simulink model "rs_tlcd_predictive_control"  (R2026a)
settings: Solver=FixedStepDiscrete  StartTime=0  StopTime=pc_tstop  FixedStep=0.01
settings Model: Creator=cys  LastModifiedBy=cys
settings DebuggingCC: AlgebraicLoopMsg=error

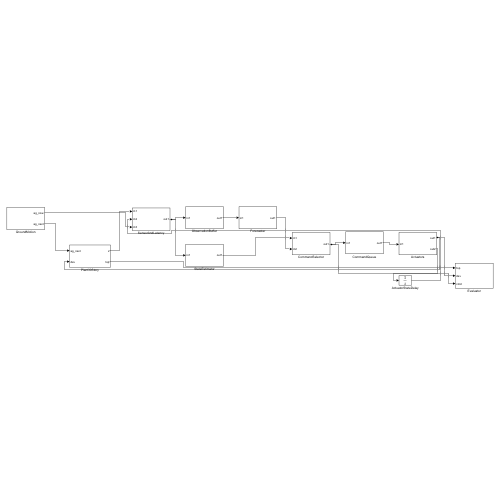
[thumbnail: Simulink's stored preview of the top-level diagram]
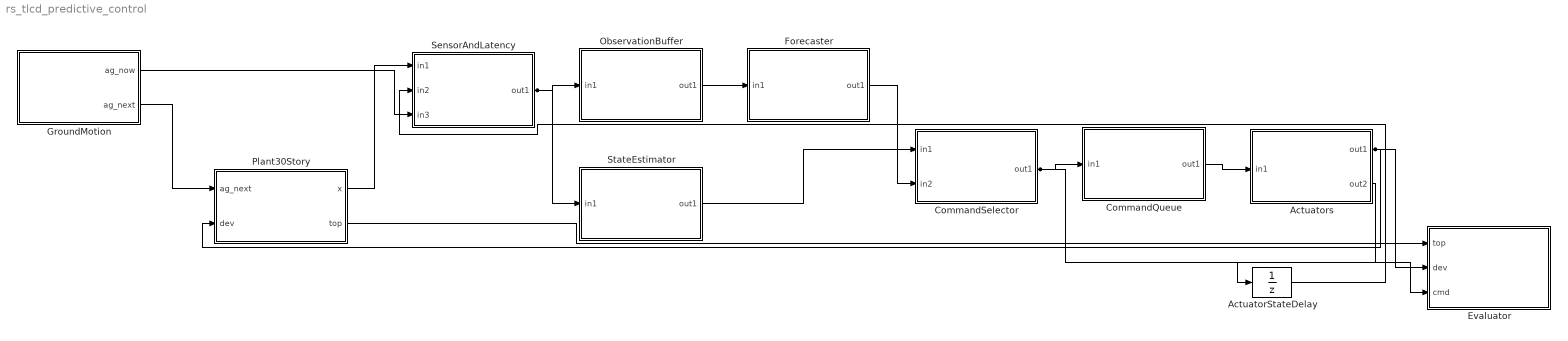
== system rs_tlcd_predictive_control ==
  ActuatorStateDelay : UnitDelay  InitialCondition=[0.3373;0;0;0.4;0.3373;0;0;0.3373;0.3373]  SampleTime=0.01
  Actuators : Subsystem
  CommandQueue : Subsystem
  CommandSelector : Subsystem
  Evaluator : Subsystem
  Forecaster : Subsystem
  GroundMotion : Subsystem
  ObservationBuffer : Subsystem
  Plant30Story : Subsystem
  SensorAndLatency : Subsystem
  StateEstimator : Subsystem
  wires:
  GroundMotion/2(ag_next) -> Plant30Story/1(ag_next)
  Actuators/1(out1) -> Plant30Story/2(dev), Evaluator/2(dev)
  Plant30Story/1(x) -> SensorAndLatency/1(in1)
  ActuatorStateDelay/1 -> SensorAndLatency/2(in2)
  GroundMotion/1(ag_now) -> SensorAndLatency/3(in3)
  SensorAndLatency/1(out1) -> ObservationBuffer/1(in1), StateEstimator/1(in1)
  ObservationBuffer/1(out1) -> Forecaster/1(in1)
  StateEstimator/1(out1) -> CommandSelector/1(in1)
  Forecaster/1(out1) -> CommandSelector/2(in2)
  CommandSelector/1(out1) -> CommandQueue/1(in1), Evaluator/3(cmd)
  CommandQueue/1(out1) -> Actuators/1(in1)
  Actuators/2(out2) -> ActuatorStateDelay/1
  Plant30Story/2(top) -> Evaluator/1(top)

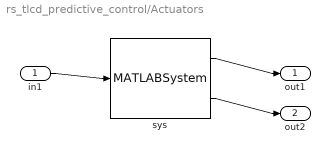
== system rs_tlcd_predictive_control/Actuators ==
  in1 : Inport
  sys : MATLABSystem  System=PCActuator  CtxVar=pc_ctx  Ts=0.01  SimulateUsing=Interpreted execution
      mask Type: PCActuator
  out1 : Outport
  out2 : Outport  Port=2
  wires:
  in1/1 -> sys/1
  sys/1 -> out1/1
  sys/2 -> out2/1

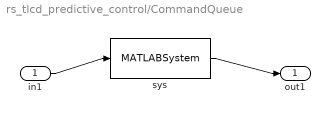
== system rs_tlcd_predictive_control/CommandQueue ==
  in1 : Inport
  sys : MATLABSystem  System=PCQueue  CtxVar=pc_ctx  Ts=0.01  SimulateUsing=Interpreted execution
      mask Type: PCQueue
  out1 : Outport
  wires:
  in1/1 -> sys/1
  sys/1 -> out1/1

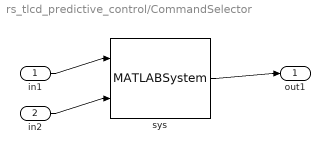
== system rs_tlcd_predictive_control/CommandSelector ==
  in1 : Inport
  in2 : Inport  Port=2
  sys : MATLABSystem  System=PCSelector  CtxVar=pc_ctx  Ts=0.01  SimulateUsing=Interpreted execution
      mask Type: PCSelector
  out1 : Outport
  wires:
  in1/1 -> sys/1
  in2/1 -> sys/2
  sys/1 -> out1/1

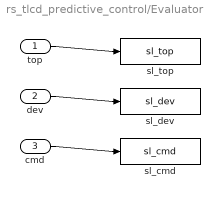
== system rs_tlcd_predictive_control/Evaluator ==
  top : Inport
  dev : Inport  Port=2
  cmd : Inport  Port=3
  sl_cmd : ToWorkspace  VariableName=sl_cmd  SampleTime=0.01
  sl_dev : ToWorkspace  VariableName=sl_dev  SampleTime=0.01
  sl_top : ToWorkspace  VariableName=sl_top  SampleTime=0.01
  wires:
  top/1 -> sl_top/1
  dev/1 -> sl_dev/1
  cmd/1 -> sl_cmd/1

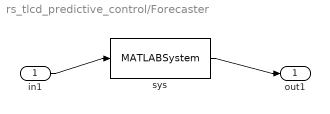
== system rs_tlcd_predictive_control/Forecaster ==
  in1 : Inport
  sys : MATLABSystem  System=PCForecaster  CtxVar=pc_ctx  Ts=0.01  SimulateUsing=Interpreted execution
      mask Type: PCForecaster
  out1 : Outport
  wires:
  in1/1 -> sys/1
  sys/1 -> out1/1

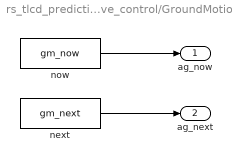
== system rs_tlcd_predictive_control/GroundMotion ==
  next : FromWorkspace  VariableName=gm_next  SampleTime=0.01  Interpolate=off  OutputAfterFinalValue=Holding final value
  now : FromWorkspace  VariableName=gm_now  SampleTime=0.01  Interpolate=off  OutputAfterFinalValue=Holding final value
  ag_now : Outport
  ag_next : Outport  Port=2
  wires:
  now/1 -> ag_now/1
  next/1 -> ag_next/1

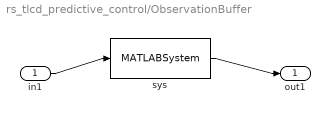
== system rs_tlcd_predictive_control/ObservationBuffer ==
  in1 : Inport
  sys : MATLABSystem  System=PCBuffer  CtxVar=pc_ctx  Ts=0.01  SimulateUsing=Interpreted execution
      mask Type: PCBuffer
  out1 : Outport
  wires:
  in1/1 -> sys/1
  sys/1 -> out1/1

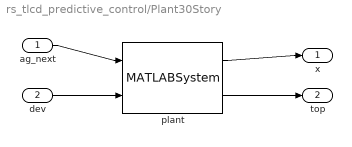
== system rs_tlcd_predictive_control/Plant30Story ==
  ag_next : Inport
  dev : Inport  Port=2
  plant : MATLABSystem  System=PCPlant  CtxVar=pc_ctx  Ts=0.01  SimulateUsing=Interpreted execution
      mask Type: PCPlant
  x : Outport
  top : Outport  Port=2
  wires:
  ag_next/1 -> plant/1
  dev/1 -> plant/2
  plant/1 -> x/1
  plant/2 -> top/1

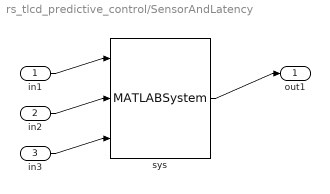
== system rs_tlcd_predictive_control/SensorAndLatency ==
  in1 : Inport
  in2 : Inport  Port=2
  in3 : Inport  Port=3
  sys : MATLABSystem  System=PCSensor  CtxVar=pc_ctx  Ts=0.01  SimulateUsing=Interpreted execution
      mask Type: PCSensor
  out1 : Outport
  wires:
  in1/1 -> sys/1
  in2/1 -> sys/2
  in3/1 -> sys/3
  sys/1 -> out1/1

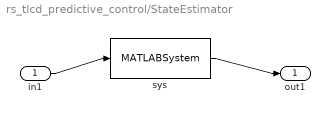
== system rs_tlcd_predictive_control/StateEstimator ==
  in1 : Inport
  sys : MATLABSystem  System=PCEstimator  CtxVar=pc_ctx  Ts=0.01  SimulateUsing=Interpreted execution
      mask Type: PCEstimator
  out1 : Outport
  wires:
  in1/1 -> sys/1
  sys/1 -> out1/1
